simulink model "atlas_docking_fsm"  (R2025a)
settings: Solver=FixedStepDiscrete  StartTime=0.0  StopTime=30  FixedStep=0.01  RelTol=1e-3
model workspace (MAT data in the model file):
  RETRY_LIMIT = 3
settings Model: Creator=mdsazzadhossain  LastModifiedBy=mdsazzadhossain

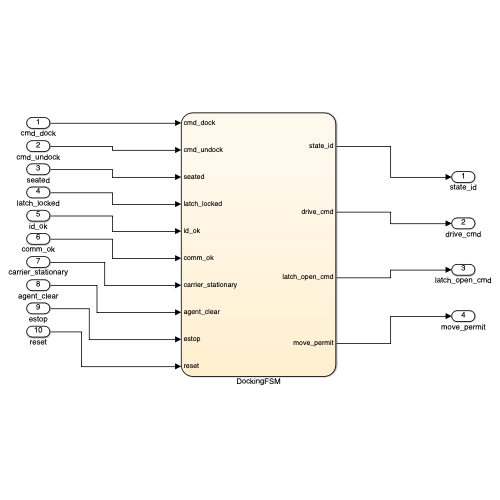
[thumbnail: Simulink's stored preview of the top-level diagram]
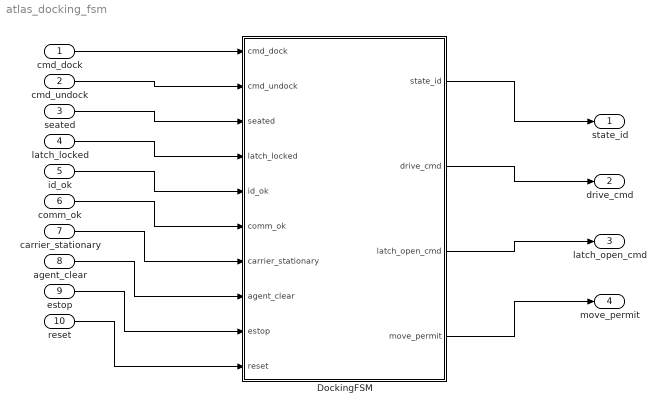
== system atlas_docking_fsm ==
  cmd_dock : Inport  OutDataTypeStr=boolean
  cmd_undock : Inport  Port=2  OutDataTypeStr=boolean
  seated : Inport  Port=3  OutDataTypeStr=boolean
  latch_locked : Inport  Port=4  OutDataTypeStr=boolean
  id_ok : Inport  Port=5  OutDataTypeStr=boolean
  comm_ok : Inport  Port=6  OutDataTypeStr=boolean
  carrier_stationary : Inport  Port=7  OutDataTypeStr=boolean
  agent_clear : Inport  Port=8  OutDataTypeStr=boolean
  estop : Inport  Port=9  OutDataTypeStr=boolean
  reset : Inport  Port=10  OutDataTypeStr=boolean
  DockingFSM : Stateflow chart  TreatAsAtomicUnit=on
  state_id : Outport
  drive_cmd : Outport  Port=2
  latch_open_cmd : Outport  Port=3
  move_permit : Outport  Port=4
  wires:
  cmd_dock/1 -> DockingFSM/1(cmd_dock)
  cmd_undock/1 -> DockingFSM/2(cmd_undock)
  seated/1 -> DockingFSM/3(seated)
  latch_locked/1 -> DockingFSM/4(latch_locked)
  id_ok/1 -> DockingFSM/5(id_ok)
  comm_ok/1 -> DockingFSM/6(comm_ok)
  carrier_stationary/1 -> DockingFSM/7(carrier_stationary)
  agent_clear/1 -> DockingFSM/8(agent_clear)
  estop/1 -> DockingFSM/9(estop)
  reset/1 -> DockingFSM/10(reset)
  DockingFSM/1(state_id) -> state_id/1
  DockingFSM/2(drive_cmd) -> drive_cmd/1
  DockingFSM/3(latch_open_cmd) -> latch_open_cmd/1
  DockingFSM/4(move_permit) -> move_permit/1

== stateflow chart atlas_docking_fsm/DockingFSM ==
  settings: updateMethod=DISCRETE  sampleTime=0.01
  state ACTIVE
    state IDLE
      entry: state_id=0; drive_cmd=0; latch_open_cmd=false; move_permit=false;
    state APPROACH
      entry: state_id=1; drive_cmd=1; latch_open_cmd=true; move_permit=false;
    state LATCHING
      entry: state_id=2; drive_cmd=0; latch_open_cmd=false;
    state VERIFY
      entry: state_id=3; drive_cmd=0;
    state BACKOFF
      entry: state_id=7; latch_open_cmd=true; drive_cmd=0; retries=retries+1;
      during: if ~latch_locked, drive_cmd=-1; else, drive_cmd=0; end
    state DOCKED
      entry: state_id=4; drive_cmd=0; latch_open_cmd=false;
      during: move_permit = seated && latch_locked;
      exit: move_permit=false;
    state RELEASING
      entry: state_id=6; drive_cmd=-1;
    state UNLATCHING
      entry: state_id=5; latch_open_cmd=true; move_permit=false;
    RELEASING -> IDLE [order 1] : [~seated && agent_clear]
    (default) -> IDLE
    LATCHING -> BACKOFF [order 2] : [~seated || after(2,sec)]
    VERIFY -> BACKOFF [order 2] : after(3,sec)
    IDLE -> APPROACH : [cmd_dock && carrier_stationary]{retries=0;}
    BACKOFF -> APPROACH [order 2] : [~seated && after(3,sec) && retries < RETRY_LIMIT]
    APPROACH -> LATCHING [order 1] : [seated]
    LATCHING -> VERIFY [order 1] : [seated && latch_locked]
    VERIFY -> DOCKED [order 1] : [seated && latch_locked && id_ok && comm_ok]
    APPROACH -> BACKOFF [order 2] : after(15,sec)
    DOCKED -> UNLATCHING [order 1] : [cmd_undock && carrier_stationary]
    UNLATCHING -> RELEASING [order 1] : [~latch_locked]
  state FAULT
    entry: state_id=9; drive_cmd=0; latch_open_cmd=false; move_permit=false;
  (default) -> ACTIVE
  FAULT -> ACTIVE : [reset && ~estop]
  BACKOFF -> FAULT [order 1] : [~seated && after(3,sec) && retries >= RETRY_LIMIT]
  BACKOFF -> FAULT [order 3] : after(10,sec)
  RELEASING -> FAULT [order 2] : after(10,sec)
  UNLATCHING -> FAULT [order 2] : after(2,sec)
  DOCKED -> FAULT [order 2] : [~seated || ~latch_locked]
  ACTIVE -> FAULT : [estop]
  data: cmd_dock input boolean; cmd_undock input boolean; seated input boolean; latch_locked input boolean; id_ok input boolean; comm_ok input boolean; carrier_stationary input boolean; agent_clear input boolean; estop input boolean; reset input boolean; state_id output double; drive_cmd output double; latch_open_cmd output boolean; move_permit output boolean; retries local double =0; RETRY_LIMIT parameter double
